simulink model "Quadri_Victor_combination_PID_R2025a"  (R2025a)
settings: Solver=FixedStepDiscrete  StartTime=0.0  StopTime=quad_t_stop  FixedStep=pid_dt  RelTol=1e-3  EnableMultiTasking=on
InitFcn:
  | run(fullfile(fileparts(fileparts(get_param(bdroot,'FileName'))),'params','victor_pid_params.m'))
undefined symbols (not defined in the file): pid_dt, quad_int0, quad_param_vec, quad_x0
settings Model: ExtModeTrigDuration=10000  Creator=gandhico  LastModifiedBy=gandhico
settings SolverCC: AlgebraicLoopSolver=TrustRegion  PositivePriorityOrder=on
settings DataIOCC: ReturnWorkspaceOutputs=off
settings DebuggingCC: UnconnectedInputMsg=warning  UnconnectedOutputMsg=warning  UnconnectedLineMsg=warning  ArithmeticOperatorsInVariantConditions=warning
settings ModelReferenceCC: EnableRefExpFcnMdlSchedulingChecks=on
settings SFSimCC: SimUseLocalCustomCode=off  CustomCodeUndefinedFunction=UseInterfaceOnly
settings RTWCC: RTWUseLocalCustomCode=off  Toolchain=QUARC win64 | nmake (64-bit Windows)  BuildConfiguration=Faster Runs  GPUComputeCapability=3.5
settings CodeAppCC: StateflowObjectComments=on
settings ConfigComp: CovMetricSettings=dswe

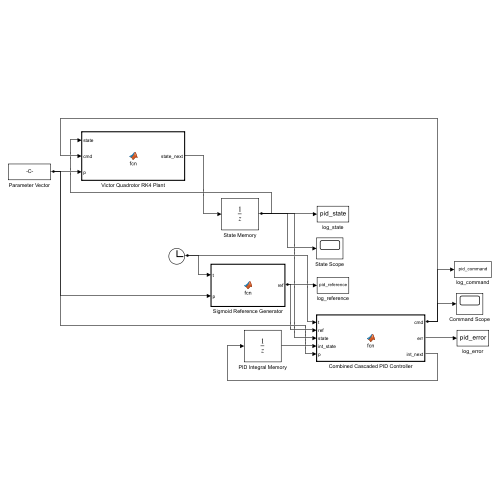
[thumbnail: Simulink's stored preview of the top-level diagram]
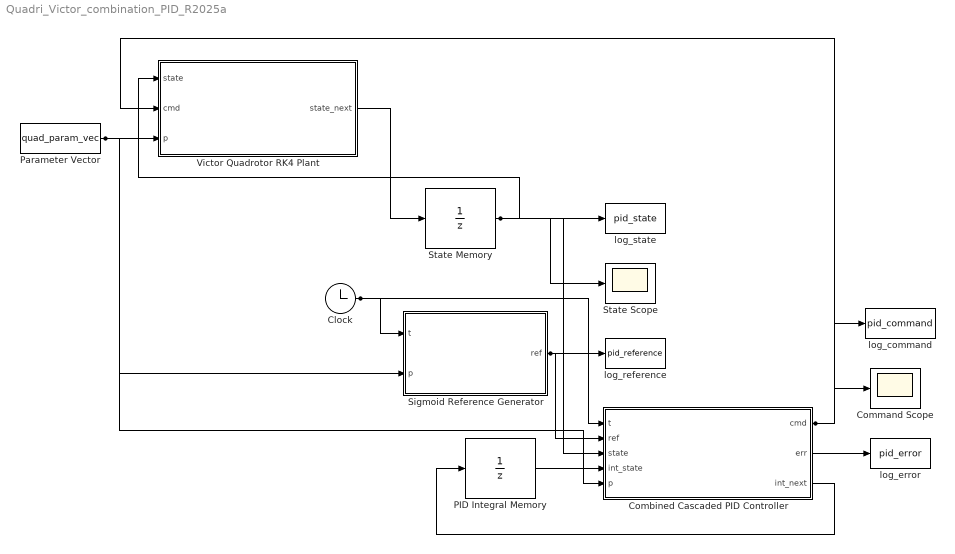
== system Quadri_Victor_combination_PID_R2025a ==
  Clock : Clock
  Combined Cascaded PID Controller : MATLAB Function  TreatAsAtomicUnit=on
  Command Scope : Scope
  PID Integral Memory : UnitDelay  InitialCondition=quad_int0  SampleTime=pid_dt  HasFrameUpgradeWarning=on
  Parameter Vector : Constant  Value=quad_param_vec
  Sigmoid Reference Generator : MATLAB Function  TreatAsAtomicUnit=on
  State Memory : UnitDelay  InitialCondition=quad_x0  SampleTime=pid_dt  HasFrameUpgradeWarning=on
  State Scope : Scope
  Victor Quadrotor RK4 Plant : MATLAB Function  TreatAsAtomicUnit=on
  log_command : ToWorkspace  VariableName=pid_command  SaveFormat=Structure With Time  SampleTime=-1
  log_error : ToWorkspace  VariableName=pid_error  SaveFormat=Structure With Time  SampleTime=-1
  log_reference : ToWorkspace  VariableName=pid_reference  SaveFormat=Structure With Time  SampleTime=-1
  log_state : ToWorkspace  VariableName=pid_state  SaveFormat=Structure With Time  SampleTime=-1
  wires:
  Parameter Vector/1 -> Sigmoid Reference Generator/2(p), Combined Cascaded PID Controller/5(p), Victor Quadrotor RK4 Plant/3(p)
  Clock/1 -> Combined Cascaded PID Controller/1(t), Sigmoid Reference Generator/1(t)
  Victor Quadrotor RK4 Plant/1(state_next) -> State Memory/1
  Combined Cascaded PID Controller/1(cmd) -> log_command/1, Victor Quadrotor RK4 Plant/2(cmd), Command Scope/1
  PID Integral Memory/1 -> Combined Cascaded PID Controller/4(int_state)
  State Memory/1 -> Victor Quadrotor RK4 Plant/1(state), Combined Cascaded PID Controller/3(state), log_state/1, State Scope/1
  Sigmoid Reference Generator/1(ref) -> Combined Cascaded PID Controller/2(ref), log_reference/1
  Combined Cascaded PID Controller/2(err) -> log_error/1
  Combined Cascaded PID Controller/3(int_next) -> PID Integral Memory/1

== matlab function Quadri_Victor_combination_PID_R2025a/Combined Cascaded PID Controller ==
  data: t input size=[1 1]; cmd output size=[9 1]; ref input size=[7 1]; state input size=[12 1]; int_state input size=[6 1]; p input size=[36 1]; err output size=[12 1]; int_next output size=[6 1]
function [cmd, err, int_next] = fcn(t, ref, state, int_state, p)
%#codegen
pid_dt = p(1);
m = p(2);
g = p(3);
kp_z = p(9); ki_z = p(10); kd_z = p(11);
kp_x = p(12); ki_x = p(13); kd_x = p(14);
kp_y = p(15); ki_y = p(16); kd_y = p(17);
kp_psi = p(18); ki_psi = p(19); kd_psi = p(20);
kp_theta = p(21); ki_theta = p(22); kd_theta = p(23);
kp_phi = p(24); ki_phi = p(25); kd_phi = p(26);
tilt_limit = p(27);
den_min = p(28);
u_min = p(29);
u_max = p(30);
tau_psi_limit = p(31);
tau_theta_limit = p(32);
tau_phi_limit = p(33);
int_xy_lim = p(34);
int_z_lim = p(35);
int_att_lim = p(36);

x = state(1); dx = state(2);
y = state(3); dy = state(4);
z = state(5); dz = state(6);
psi = state(7); dpsi = state(8);
theta = state(9); dtheta = state(10);
phi = state(11); dphi = state(12);

ex = ref(1) - x;
edx = ref(2) - dx;
ey = ref(3) - y;
edy = ref(4) - dy;
ez = ref(5) - z;
edz = -dz;
epsi = wrap_pi(ref(7) - psi);
edpsi = -dpsi;

integ_new = int_state;
integ_new(1) = sat(int_state(1) + pid_dt*ex, int_xy_lim);
integ_new(2) = sat(int_state(2) + pid_dt*ey, int_xy_lim);
integ_new(3) = sat(int_state(3) + pid_dt*ez, int_z_lim);
integ_new(4) = sat(int_state(4) + pid_dt*epsi, int_att_lim);

ax_cmd = kp_x*ex + ki_x*integ_new(1) + kd_x*edx;
ay_cmd = kp_y*ey + ki_y*integ_new(2) + kd_y*edy;
uz_cmd = kp_z*ez + ki_z*integ_new(3) + kd_z*edz;

theta_d = atan2(ax_cmd, g);
phi_d = atan2(-ay_cmd*cos(theta), g);
theta_d = sat(theta_d, tilt_limit);
phi_d = sat(phi_d, tilt_limit);

etheta = theta_d - theta;
edtheta = -dtheta;
ephi = phi_d - phi;
edphi = -dphi;
integ_new(5) = sat(int_state(5) + pid_dt*etheta, int_att_lim);
integ_new(6) = sat(int_state(6) + pid_dt*ephi, int_att_lim);

u_unsat = (m*g + uz_cmd)/max(cos(theta)*cos(phi), den_min);
u = min(max(u_unsat, u_min), u_max);

tau_psi_unsat = kp_psi*epsi + ki_psi*integ_new(4) + kd_psi*edpsi;
tau_theta_unsat = kp_theta*etheta + ki_theta*integ_new(5) + kd_theta*edtheta;
tau_phi_unsat = kp_phi*ephi + ki_phi*integ_new(6) + kd_phi*edphi;

tau_psi = sat(tau_psi_unsat, tau_psi_limit);
tau_theta = sat(tau_theta_unsat, tau_theta_limit);
tau_phi = sat(tau_phi_unsat, tau_phi_limit);

cmd = [u; tau_psi; tau_theta; tau_phi; theta_d; phi_d; ax_cmd; ay_cmd; uz_cmd];
err = [ex; ey; ez; epsi; etheta; ephi; integ_new(1); integ_new(2); integ_new(3); integ_new(4); integ_new(5); integ_new(6)];
int_next = integ_new;
end

function y = sat(x, lim)
y = min(max(x, -lim), lim);
end

function y = wrap_pi(x)
y = mod(x + pi, 2*pi) - pi;
end

== matlab function Quadri_Victor_combination_PID_R2025a/Sigmoid Reference Generator ==
  data: t input size=[1 1]; ref output size=[7 1]; p input size=[36 1]
function ref = fcn(t, p)
%#codegen
k = p(4);
z_amp = p(5);
x_amp = p(6);
y_amp = p(7);
psi_ref_value = p(8);

% --- Sigmoid trajectory mission ----------------------------------------
%   x_d(t) = x_amp / (1 + exp(-k*(t - 5)))                  center 5, no delay
%   z_d(t) = z_amp / (1 + exp(-k*(t - 4)))                  center 4, no delay
%   y_d(t) = 0                              for t <  y_delay
%          = y_amp / (1 + exp(-k*((t - y_delay) - 5)))      center 5, delayed
% Amplitudes (x_amp, y_amp, z_amp) and k come from params/victor_pid_params.m;
% the centers and the y-channel delay are defined here.
y_delay = 15.0;

[z_ref, dz_sigmoid] = sigmoid_ref(t, z_amp, k, 4.0);
[x_ref, dx_ref] = sigmoid_ref(t, x_amp, k, 5.0);
if t < y_delay
    y_ref = 0.0;
    dy_ref = 0.0;
else
    [y_ref, dy_ref] = sigmoid_ref(t - y_delay, y_amp, k, 5.0);
end

% The original Victor Fcn z controller damps measured dz only; it does not
% subtract dz_ref. Keep this channel zero to make that convention explicit.
dz_ref = 0.0;
psi_ref = psi_ref_value;
ref = [x_ref; dx_ref; y_ref; dy_ref; z_ref; dz_ref; psi_ref];
end

function [r, dr] = sigmoid_ref(t, amp, k, center)
q = exp(-k*(t - center));
den = 1.0 + q;
r = amp/den;
dr = amp*k*q/(den*den);
end

== matlab function Quadri_Victor_combination_PID_R2025a/Victor Quadrotor RK4 Plant ==
  data: state input size=[12 1]; state_next output size=[12 1]; cmd input size=[9 1]; p input size=[36 1]
function state_next = fcn(state, cmd, p)
%#codegen
h = p(1);
k1 = dyn_quad(state, cmd, p);
k2 = dyn_quad(state + 0.5*h*k1, cmd, p);
k3 = dyn_quad(state + 0.5*h*k2, cmd, p);
k4 = dyn_quad(state + h*k3, cmd, p);
state_next = state + (h/6.0)*(k1 + 2.0*k2 + 2.0*k3 + k4);
end

function dX = dyn_quad(x, cmd, p)
m = p(2);
g = p(3);
u = cmd(1);
tau_psi = cmd(2);
tau_theta = cmd(3);
tau_phi = cmd(4);
psi = x(7); theta = x(9); phi = x(11);

dX = zeros(12,1);
dX(1) = x(2);
dX(2) = u*(sin(phi)*sin(psi) + cos(phi)*cos(psi)*sin(theta))/m;
dX(3) = x(4);
dX(4) = u*(cos(phi)*sin(theta)*sin(psi) - cos(psi)*sin(phi))/m;
dX(5) = x(6);
dX(6) = u*(cos(theta)*cos(phi))/m - g;
dX(7) = x(8);
dX(8) = tau_psi;
dX(9) = x(10);
dX(10) = tau_theta;
dX(11) = x(12);
dX(12) = tau_phi;
end
